simulink model "sns_tutorial2_twin"  (R2025a)
settings: Solver=ode45  StartTime=0.0  StopTime=0.05  RelTol=1e-8  AbsTol=1e-10
libraries: SNS_Library x11
settings Model: Creator=Ben Bolen  LastModifiedBy=Ben Bolen
settings DataIOCC: SignalLoggingName=sigs

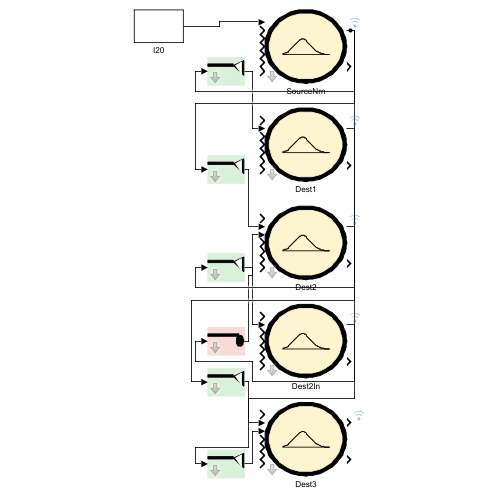
[thumbnail: Simulink's stored preview of the top-level diagram]
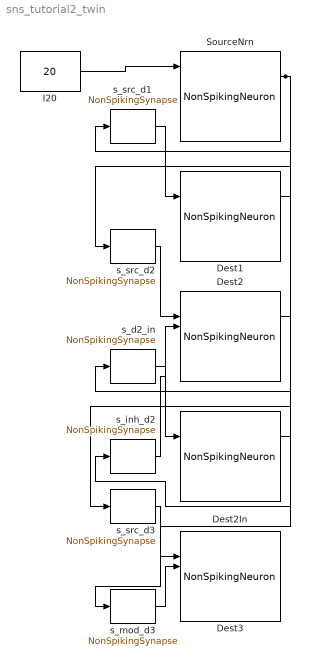
== system sns_tutorial2_twin ==
  Dest1 : SNS_Library/NonSpikingNeuron  Vrest=0  Gm=1  Cm=5  Thr=0  Slope=20
  Dest2 : SNS_Library/NonSpikingNeuron  Vrest=0  Gm=1  Cm=5  Thr=0  Slope=20
  Dest2In : SNS_Library/NonSpikingNeuron  Vrest=0  Gm=1  Cm=5  Thr=0  Slope=20
  Dest3 : SNS_Library/NonSpikingNeuron  Vrest=0  Gm=1  Cm=5  Thr=0  Slope=20
  I20 : Constant  Value=20
  SourceNrn : SNS_Library/NonSpikingNeuron  Vrest=0  Gm=1  Cm=5  Thr=0  Slope=20
  s_d2_in : SNS_Library/NonSpikingSynapse  gmax=1  Esyn=50  ThrPre=0  SlopePre=20
  s_inh_d2 : SNS_Library/NonSpikingSynapse  gmax=1  Esyn=-40  ThrPre=0  SlopePre=20
  s_mod_d3 : SNS_Library/NonSpikingSynapse  gmax=1  Esyn=0  ThrPre=0  SlopePre=20
  s_src_d1 : SNS_Library/NonSpikingSynapse  gmax=1  Esyn=50  ThrPre=0  SlopePre=20
  s_src_d2 : SNS_Library/NonSpikingSynapse  gmax=1  Esyn=50  ThrPre=0  SlopePre=20
  s_src_d3 : SNS_Library/NonSpikingSynapse  gmax=1  Esyn=50  ThrPre=0  SlopePre=20
  wires:
  I20/1 -> SourceNrn/1
  SourceNrn/1 -> s_src_d1/1, s_src_d2/1, s_src_d3/1
  s_src_d1/1 -> Dest1/2
  s_src_d2/1 -> Dest2/2
  Dest2/1 -> s_d2_in/1
  s_d2_in/1 -> Dest2In/2
  Dest2In/1 -> s_inh_d2/1
  s_inh_d2/1 -> Dest2/3
  s_src_d3/1 -> Dest3/2
  Dest1/1 -> s_mod_d3/1
  s_mod_d3/1 -> Dest3/3
